simulink model "Controller_jtorque_cbf_22Franka"  (R2022b)
settings: Solver=FixedStepDiscrete  StartTime=0.0  StopTime=inf  FixedStep=0.001  RelTol=1e-3
PreLoadFcn:
  | set_param(gcs, 'RTWSystemTargetFile', 'franka_emika_panda.tlc');
  | 
  | demos_common_configs();
  | collision_behavior = ones(1,52)*100;
values from neighbouring files (symbols this model uses):
  b_sg = fliplr(B(end, :))    [init_joint_torque_cbf.m]
  cbf_dt = 0.001    [init_joint_torque_cbf.m]
  cbf_jtorque_params = [cbf_p_ths; cbf_v_ths; cbf_v_0; cbf_gamma; cbf_w_lin; cbf_w_slack;                        cbf_tau_limit; cbf_dt; plane_normal; plane_offset;                        cbf_latch_entry; cbf_zone_hyst; cbf_latch_alpha; cbf_tau_max;                        cbf_tau_rate; cbf_max_lat_force; cbf_max_moment;                        cbf_w_lateral; cbf_w_moment; cbf_w_null; cbf_guar_factor]    [init_joint_torque_cbf.m]
  cbf_Kd_rot = [120; 120; 120]*0    [init_joint_torque_cbf.m]
  cbf_Kd_trans = [2000; 2000; 0]*0    [init_joint_torque_cbf.m]
  cbf_stiff_decouple = 0    [init_joint_torque_cbf.m]
  cbf_zeta_rot = [0.7; 0.7; 0.7]*0    [init_joint_torque_cbf.m]
  cbf_zeta_trans = [0.7; 0.7; 0]*0    [init_joint_torque_cbf.m]
  Dn = 0 * ones(7,1)    [init_joint_torque_cbf.m]
  H_home = getTransform(Franka_robot, q_home, 'panda_link8', 'panda_link0')    [init_joint_torque_cbf.m]
  Kn = 0 * ones(7,1)    [init_joint_torque_cbf.m]
  plane_normal = [0.0; 0.0; 1.0]    [init_joint_torque_cbf.m]
  q_home = q_init    [init_joint_torque_cbf.m]
  q_init = [0 0  0  -(2/4)*pi  0  pi/2  -pi/4]'    [init_joint_torque_cbf.m]
undefined symbols (not defined in the file or in its folder): DiscIntNeverNeededParam, Fext_mag
libraries: franka_simulink_library x2, Robotics_lib x1, matrix_library x1
(part 5 of 7)

== matlab function Controller_jtorque_cbf_22Franka/task space controller/Lateral_Stiffness ==
  data: H_I_t input; tau_stiff output; H_I_D input; Jg input; KdTrans input; KdRot input; q_dot input; Lambda input; ZetaTrans input; ZetaRot input; n_hp input; decouple input
function tau_stiff = fcn(H_I_t, H_I_D, Jg, KdTrans, KdRot, q_dot, Lambda, ZetaTrans, ZetaRot, n_hp, decouple)
%% Cartesian spring-damper torque (no Coriolis / feed-forward terms).
%% Spring as Stiffnessforces/MATLAB Function3 of the damping model:
%%   Fk = [KdTrans*(x - x_D); 2*R_D*(eta*I + skew(eps))*KdRot*eps]
%% Damping with constant damping ratio (Lambda = Cartesian mass matrix):
%%   Fd = D .* (Jg*q_dot),  D_i = 2*zeta_i*sqrt(K_i*Lambda_ii)
%% Decoupling from the plane normal n6 (decouple = 1):
%%   F = F - n6*(n6'*Lambda^-1*F)/(n6'*Lambda^-1*n6)  -> zero acceleration along n6
%%   tau = -Jg'*F
lam = diag(Lambda);
Dtrans = 2.*ZetaTrans(:).*sqrt(KdTrans(:).*max(lam(1:3), 0));
Drot   = 2.*ZetaRot(:).*sqrt(KdRot(:).*max(lam(4:6), 0));
V = Jg*q_dot;
Fd = [Dtrans.*V(1:3); Drot.*V(4:6)];

KdTrans = diag(KdTrans);
KdRot = diag(KdRot);

R_D_t = (H_I_D(1:3,1:3))'*H_I_t(1:3,1:3);

eta_D_t = 0.5*sqrt(abs(1 + R_D_t(1,1) + R_D_t(2,2) + R_D_t(3,3)));
epsi_D_t = 0.5.*[MySign(R_D_t(3,2) - R_D_t(2,3))*realsqrt(abs( R_D_t(1,1)-R_D_t(2,2)-R_D_t(3,3)+1));
                 MySign(R_D_t(1,3) - R_D_t(3,1))*realsqrt(abs(-R_D_t(1,1)+R_D_t(2,2)-R_D_t(3,3)+1));
                 MySign(R_D_t(2,1) - R_D_t(1,2))*realsqrt(abs(-R_D_t(1,1)-R_D_t(2,2)+R_D_t(3,3)+1))];

epsi_D_t_skew = [0,           -epsi_D_t(3),  epsi_D_t(2);
                 epsi_D_t(3),   0,           -epsi_D_t(1);
                -epsi_D_t(2),   epsi_D_t(1),  0];

x_tilde = H_I_t(1:3,4) - H_I_D(1:3,4);

Fktrans = KdTrans*x_tilde;
Fkrot = 2.*H_I_D(1:3,1:3)*(eta_D_t.*eye(3) + epsi_D_t_skew)*KdRot*epsi_D_t;
Fk = [Fktrans; Fkrot];
F = Fk + Fd;

if decouple > 0.5
    n6 = n_hp(:);
    n6 = n6 ./ norm(n6);
    Lambda_inv = Lambda \ eye(6);
    Lambda_inv = 0.5.*(Lambda_inv + transpose(Lambda_inv));
    a_n = transpose(n6)*Lambda_inv*F;          %% normal acceleration caused by F
    c_n = transpose(n6)*Lambda_inv*n6;         %% = 1/rho along the normal
    F = F - n6.*(a_n/c_n);
end

tau_stiff = -transpose(Jg)*F;
end

function x = MySign(val)
%% sign function with MySign(0) = 1 (Siciliano 2010, eq. 2.35)
x = 1;
if (val < 0)
    x = -1;
end
end

== matlab function Controller_jtorque_cbf_22Franka/Franka Forward Dynamics /MATLAB Function ==
  data: wrench input; force output
function force = fcn(wrench)

force = wrench(1:3);

end

== matlab function Controller_jtorque_cbf_22Franka/MATLAB Function ==
  data: H input; p output
function p = fcn(H)

p = H(1:3,4);

== matlab function Controller_jtorque_cbf_22Franka/task space controller/MATLAB Function1 ==
  data: n_hp input; F_ext output; wrench_ext input
function F_ext = fcn(n_hp, wrench_ext)

% F_ext = (n_hp).*wrench_ext;
F_ext = wrench_ext;

end

== matlab function Controller_jtorque_cbf_22Franka/MATLAB Function2 ==
  data: H_init input; H_ref output; d input; R_I_t output
function [H_ref, R_I_t] = fcn(H_init, d)

H_ref = H_init;
% H_ref(1:3,4) = d;
R_I_t = H_ref(1:3,1:3);

end
